simulink model "Circuito_Simulink_acquisizione"  (R2023b)
settings: Solver=FixedStepAuto  StartTime=0.0  StopTime=60  RelTol=1e-3
libraries: androidsensorlib x2
settings Model: Creator=Marco  LastModifiedBy=Marco
settings OptimizationCC: EnhancedBackFolding=on  PassReuseOutputArgsThreshold=0  MaxStackSize=64  OptimizeBlockOrder=speed  DifferentSizesBufferReuse=on  OptimizationCustomize=off
settings DebuggingCC: ParameterTunabilityLossMsg=error
settings HardwareCC: ProdBitPerLong=64  ProdLargestAtomicInteger=LongLong  ProdLargestAtomicFloat=Double  ProdLongLongMode=on  ProdHWDeviceType=ARM Compatible->ARM 64-bit (LP64)  UseEmbeddedCoderFeatures=off  UseSimulinkCoderFeatures=off
settings SFSimCC: MATLABDynamicMemAlloc=off
settings RTWCC: Description=Embedded Coder  SystemTargetFile=ert.tlc  HardwareBoard=Android Device (64bit)  TLCOptions="-aInlineSetEventsForThisBaseRateFcn=TLC_FALSE -aSuppressMultiTaskScheduler=TLC_FALSE  -aRateBasedStepFcn=0"  TemplateMakefile=ert_default_tmf  RTWVerbose=off  Toolchain=Android SDK/NDK Tools
settings CodeAppCC: ForceParamTrailComments=on  OperatorAnnotations=on  MangleLength=10
settings ERTTargetCC: ERTCustomFileBanners=off  SupportContinuousTime=on  SupportNonInlinedSFcns=on  RemoveResetFunc=off  ModelStepFunctionPrototypeControlCompliant=off  ExtMode=on  ExtModeMexArgs='172.20.10.3' 0 17725  ERTSrcFileBannerTemplate=codertarget_code_template.cgt  ERTHdrFileBannerTemplate=codertarget_code_template.cgt  ERTDataSrcFileTemplate=codertarget_code_template.cgt  ERTDataHdrFileTemplate=codertarget_code_template.cgt

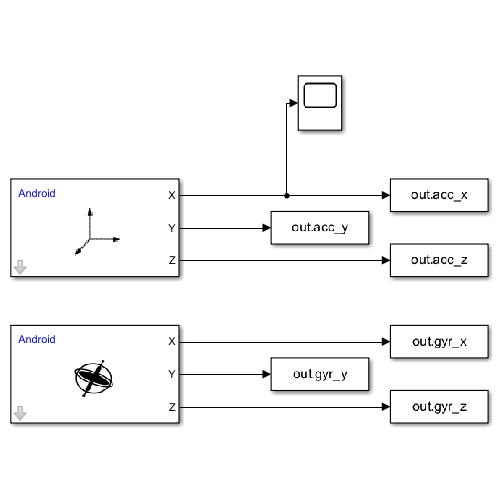
[thumbnail: Simulink's stored preview of the top-level diagram]
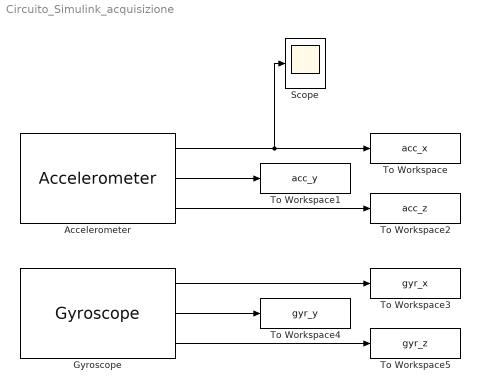
== system Circuito_Simulink_acquisizione ==
  Accelerometer : androidsensorlib/Accelerometer  OutputVector=off  SampleTime=0.005  BlockPlatform=Android
  Gyroscope : androidsensorlib/Gyroscope  OutputVector=off  SampleTime=0.005  BlockPlatform=Android
  Scope : Scope
  To Workspace : ToWorkspace  VariableName=acc_x  SaveFormat=Structure With Time  SampleTime=-1
      settings: Save2DSignal=2-D array (concatenate along first dimension)
  To Workspace1 : ToWorkspace  VariableName=acc_y  SaveFormat=Structure With Time  SampleTime=-1
      settings: Save2DSignal=2-D array (concatenate along first dimension)
  To Workspace2 : ToWorkspace  VariableName=acc_z  SaveFormat=Structure With Time  SampleTime=-1
      settings: Save2DSignal=2-D array (concatenate along first dimension)
  To Workspace3 : ToWorkspace  VariableName=gyr_x  SaveFormat=Structure With Time  SampleTime=-1
      settings: Save2DSignal=2-D array (concatenate along first dimension)
  To Workspace4 : ToWorkspace  VariableName=gyr_y  SaveFormat=Structure With Time  SampleTime=-1
      settings: Save2DSignal=2-D array (concatenate along first dimension)
  To Workspace5 : ToWorkspace  VariableName=gyr_z  SaveFormat=Structure With Time  SampleTime=-1
      settings: Save2DSignal=2-D array (concatenate along first dimension)
  wires:
  Accelerometer/2 -> To Workspace1/1
  Accelerometer/1 -> Scope/1, To Workspace/1
  Accelerometer/3 -> To Workspace2/1
  Gyroscope/1 -> To Workspace3/1
  Gyroscope/3 -> To Workspace5/1
  Gyroscope/2 -> To Workspace4/1
